simulink model "exp2"  (R2023b)
settings: Solver=VariableStepAuto  StartTime=0.0  StopTime=1  RelTol=1e-3
undefined symbols (not defined in the file): Acid, Lead
libraries: spsSeriesRLCBranchLib x3, spsBatteryLib x1, spsDiodeLib x1, spsMosfetLib x1, spsPVArrayLib x1, simulink x1, sps_lib x1
settings Model: Creator=manik  LastModifiedBy=muges

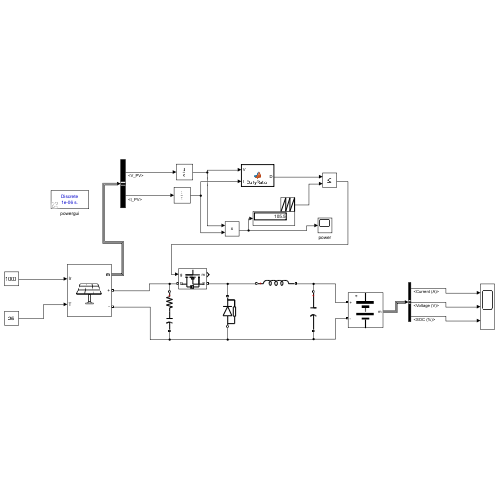
[thumbnail: Simulink's stored preview of the top-level diagram]
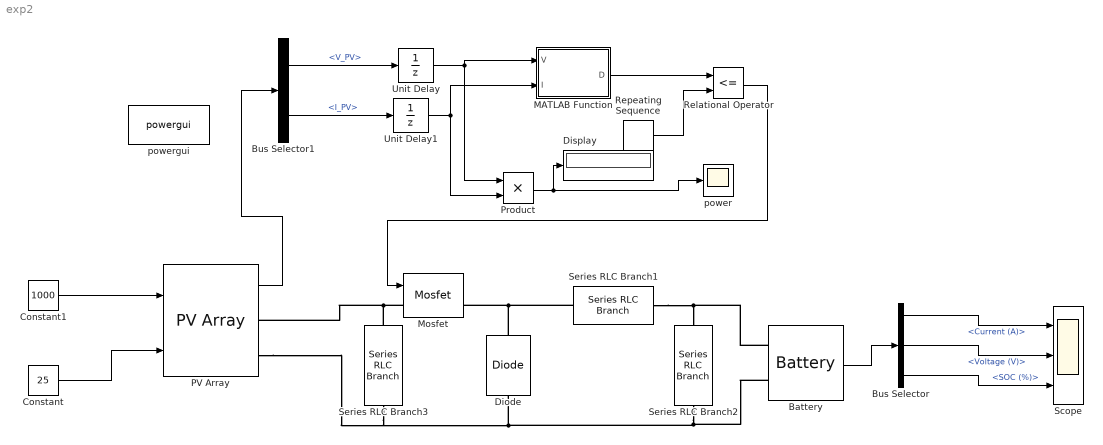
== system exp2 ==
  Battery : spsBatteryLib/Battery  BatType=Lead-Acid  ShowTempParam=off  ThermalPreset=no  ShowAgeParam=off  NomV=12  NomQ=150  SOC=45  Batt_Tr=30  PresetModel=on  MaxQ=156.25  MinV=9  FullV=13.0658  Dis_rate=30  R=0.0008  Normal_OP=46.5417  expZone="[12.2171          0.5]"  current=[6.5 13 32.5]  Units=Time  Tci=20  NomT=20  T2=-30  MaxQ2=4.8  FullV2=7.1  Normal_OP2=5.655  expZone2="[6.58           1]"  Rca=0.6  ti=2000  Dp=0  Neq0=0  Tsim=1e6  Ta1=25  Qeol=5.4*0.9  Reol=0.013333*1.2  Char_age=[2.3478, 3]  Dis_age=[2.3478, 10]  N1=1500  N2=10500  N3=1000  N4=1400  Ta2=45  N5=950
  Bus Selector : BusSelector  OutputSignals=Current (A),Voltage (V),SOC (%)
  Bus Selector1 : BusSelector  OutputSignals=V_PV,I_PV
  Constant : Constant  Value=25
  Constant1 : Constant  Value=1000
  Diode : spsDiodeLib/Diode  Ron=0.001  Lon=0  Vf=0.8  IC=0  UseSnubber=0  Rs=500  Cs=250e-9  Measurements=off
  Display : Display
  MATLAB Function : MATLAB Function  TreatAsAtomicUnit=on
  Mosfet : spsMosfetLib/Mosfet  Ron=0.1  Lon=0  Rd=0.01  Vfd=0  IC=0  Rs=1e5  Cs=inf  Measurements=on
  PV Array : spsPVArrayLib/PV Array  Npar=1  Nser=1  PlotType=array @ 1000 W/m2 & specified temperatures  S_vec="[ 1000  500  100 ]"  Temp_C_vec="[ 45 25  ]"  ModuleName=User-defined  PlotWhenSelected=off  Pm=213.15  Ncell=60  Voc=36.3  Isc=7.84  Vm=29  Im=7.35  beta_Voc_pc=-0.36099  alpha_Isc_pc=0.102  beta_Voc=-0.13104  alpha_Isc=0.0079968  IL=7.8654  I0=2.9273e-10  nI=0.98119  Rsh=313.0553  Rs=0.39381  RobustModel=off  RobustCellTemperature=313.3991  BAL=on  Tc=1e-6  Tfilter=5e-5
  Product : Product
  Relational Operator : RelationalOperator  Operator=<=  OutDataTypeStr=boolean  RndMeth=Simplest  InputSameDT=off
  Repeating Sequence : simulink/Sources/Repeating Sequence  rep_seq_t=[0 1/10000]  rep_seq_y=[0 1]
  Scope : Scope  NumInputPorts=3
  Series RLC Branch1 : spsSeriesRLCBranchLib/Series RLC Branch  LConnTagsString=__new0  RConnTagsString=__new0  BranchType=L  Resistance=1  Inductance=0.86e-3  SetiL0=off  InitialCurrent=0  Capacitance=1e-6  Setx0=off  InitialVoltage=0  Measurements=None
  Series RLC Branch2 : spsSeriesRLCBranchLib/Series RLC Branch  LConnTagsString=__new0  RConnTagsString=__new0  BranchType=C  Resistance=1  Inductance=1e-3  SetiL0=off  InitialCurrent=0  Capacitance=360e-6  Setx0=off  InitialVoltage=0  Measurements=None
  Series RLC Branch3 : spsSeriesRLCBranchLib/Series RLC Branch  LConnTagsString=__new0  RConnTagsString=__new0  BranchType=RC  Resistance=0.001  Inductance=1e-3  SetiL0=off  InitialCurrent=0  Capacitance=1000e-6  Setx0=off  InitialVoltage=0  Measurements=None
  Unit Delay : UnitDelay  SampleTime=1e-6  HasFrameUpgradeWarning=on
  Unit Delay1 : UnitDelay  SampleTime=1e-6  HasFrameUpgradeWarning=on
  power : Scope
  powergui : sps_lib/powergui  Priority=1  SimulationMode=Discrete  SampleTime=1e-6  frequency=60  Iterations=50  frequencyindice=0  Pbase=100e6  ErrMax=1e-4  UnitsV=kV  UnitsW=MW  buscounter=0  FunctionMessages=off  echomessages=off  EnableUseOfTLC=off  CurrentSourceSwitches=off  DisableSnubberDevices=off  DisableRonSwitches=off  DisableVfSwitches=off  DisplayEquations=off  AutomaticDiscreteSolvers=off  SolverType=Tustin/Backward Euler (TBE)  Interpol=off  ExternalGateDelay=off  methode=off  Ts=100  x0status=blocks  SPID=on  SwTol=0  HookPort=off  NonlinearTolerance=1e-4  nMaxIteration=100  ContinueOnMaxIteration=off  RestoreLinks=warning  ResistiveCurrentMeasurement=off  Frange=[0:2:500]  Ylog=off  Xlog=on  ShowGrid=off  save=off  variable=ZData  structure=0  ZoomFFT=off  StartTime=0.0  cycles=1  DisplayStyle=1  fundamental=60  FreqAxis=off  MaxFrequency=1000  frequencyindicesteady=1  RmsSteady=1  display=off
  wires:
  Constant/1 -> PV Array/2
  Constant1/1 -> PV Array/1
  Battery/1 -> Bus Selector/1
  Bus Selector/1 -> Scope/1  "<Current (A)>"
  Bus Selector/2 -> Scope/2  "<Voltage (V)>"
  Bus Selector/3 -> Scope/3  "<SOC (%)>"
  PV Array/1 -> Bus Selector1/1
  Bus Selector1/1 -> Unit Delay/1  "<V_PV>"
  Bus Selector1/2 -> Unit Delay1/1  "<I_PV>"
  Unit Delay/1 -> MATLAB Function/1(V), Product/1
  Unit Delay1/1 -> Product/2, MATLAB Function/2(I)
  Product/1 -> power/1, Display/1
  MATLAB Function/1(D) -> Relational Operator/1
  Repeating Sequence/1 -> Relational Operator/2
  Relational Operator/1 -> Mosfet/1
  connections:
  Series RLC Branch2/RConn1 -- Battery/LConn2 -- Series RLC Branch3/RConn1 -- PV Array/RConn2 -- Diode/LConn1
  Mosfet/LConn1 -- Series RLC Branch3/LConn1 -- PV Array/RConn1
  Diode/RConn1 -- Series RLC Branch1/LConn1 -- Mosfet/RConn1
  Battery/LConn1 -- Series RLC Branch1/RConn1 -- Series RLC Branch2/LConn1

== matlab function exp2/MATLAB Function ==
  data: V input; D output; I input
function D = DutyRatio(V, I)
    Dmax = 0.95;
    Dmin = 0.05;
    Dinit = 0.5;
    deltaD = 1e-4;
    
    persistent Vold Pold Dold;
    
    if isempty(Vold)
        Vold = 0;
        Pold = 0;
        Dold = Dinit;
    end
    
    P = V * I;
    dV = V - Vold;
    dP = P - Pold;
    
    if dP ~= 0
        if dP < 0
            if dV < 0
                D = Dold - deltaD;
            else
                D = Dold + deltaD;
            end
        else
            if dV < 0
                D = Dold + deltaD;
            else
                D = Dold - deltaD;
            end
        end
    else
        D = Dold;
    end
    
    if D >= Dmax || D <= Dmin
        D = Dold;
    end
    
    Dold = D;
    Vold = V;
    Pold = P;
end
